simulink model "hrg_tdm_residual_observer"  (R2025a)
settings: Solver=FixedStepDiscrete  StartTime=0.0  StopTime=0  FixedStep=1  RelTol=1e-3
model workspace (MAT data in the model file):
  obs.sampleCount = 1600
  obs.jointCarrierMap = [-0.00025765079673 -0.000416664414145 -0.000202686971327 -0.000334156912121 -0.000153535532759 -0.00025977175969 -0.00010978152307 -0.000192965109295 -7.10329454025e-05 -0.000133221632945 -3.69196965297e-05 -8.00532519635e-05 ... (3200 elements, 2x1600)]
  obs.lateCarrierMap = [0 0 0 0 0 0 0 0 0 0 0 0 ... (3200 elements, 2x1600)]
  obs.holdoutErrorMap = [-0.162387616405 -0.0989965810095 -0.0526141659259 -0.0196686023406 0.00277754819147 0.0171274479295 0.0253355675884 0.0289807611935 0.0293285386507 0.027384022459 0.0239368813756 0.0195993643707 ... (640000 elements, 400x1600)]
  obs.holdoutCount = 400
  obs.holdoutMean = [0.0025 0.0025 0.0025 0.0025 0.0025 0.0025 0.0025 0.0025 0.0025 0.0025 0.0025 0.0025 ... (400 elements, 1x400)]
  obs.allMask = [1 1 1 1 1 1 1 1 1 1 1 1 ... (1600 elements, 1x1600)]
  obs.lateMask = [0 0 0 0 0 0 0 0 0 0 0 0 ... (1600 elements, 1x1600)]
  obs.jointDesignOK = 1
  obs.lateDesignOK = 1
  obs.holdoutLimit = 0.00220536539639
Description:
  | 原生分时残差观测器，1600 个样本/帧，留出 RMS 门限 0.00220537 V。
settings Model: Creator=Administrator  LastModifiedBy=Administrator
settings DataIOCC: SaveTime=off

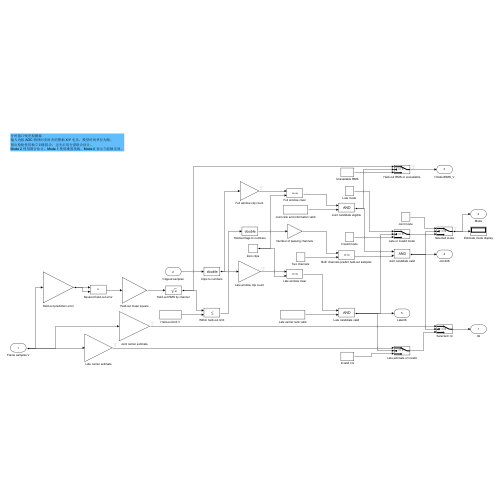
[thumbnail: Simulink's stored preview of the top-level diagram]
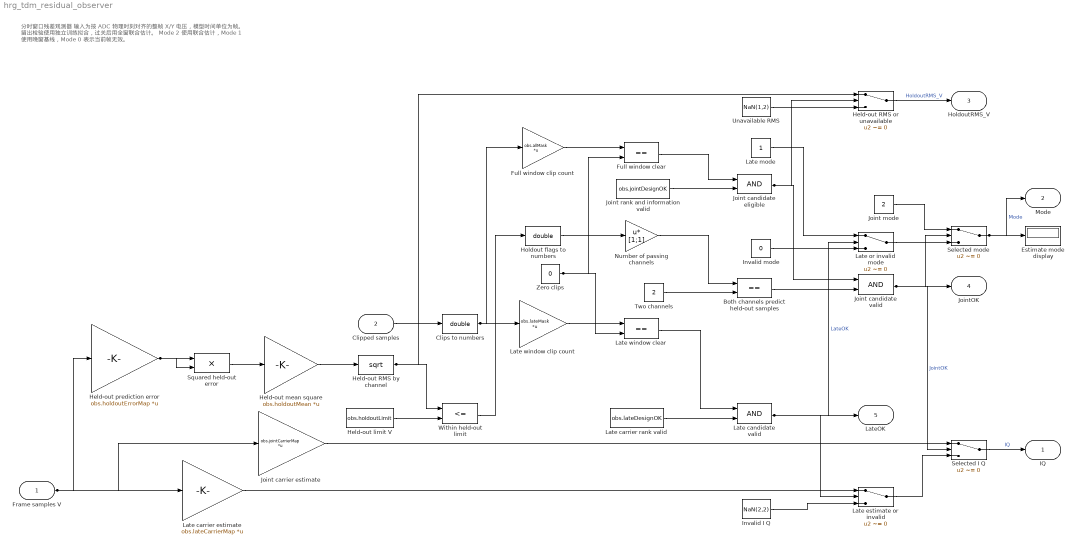
== system hrg_tdm_residual_observer ==
  note: 分时窗口残差观测器
      | 输入为按 ADC 物理时刻对齐的整帧 X/Y 电压，模型时间单位为帧。
      | 留出检验使用独立训练拟合，过关后用全窗联合估计。
      | Mode 2 使用联合估计，Mode 1 使用晚窗基线，Mode 0 表示当前帧无效。
  Frame samples V : Inport  OutDataTypeStr=double  PortDimensions=[obs.sampleCount 2]  SampleTime=1
  Clipped samples : Inport  Port=2  OutDataTypeStr=boolean  PortDimensions=obs.sampleCount  SampleTime=1
  Both channels predict held-out samples : RelationalOperator  Operator===  OutDataTypeStr=boolean  RndMeth=Simplest  InputSameDT=off
  Clips to numbers : DataTypeConversion  OutDataTypeStr=double  SaturateOnIntegerOverflow=off  RndMeth=Floor
  Estimate mode display : Display
  Full window clear : RelationalOperator  Operator===  OutDataTypeStr=boolean  RndMeth=Simplest  InputSameDT=off
  Full window clip count : Gain  Gain=obs.allMask  Multiplication=Matrix(K*u)
  Held-out RMS by channel : Math  Operator=sqrt
  Held-out RMS or unavailable : Switch  Criteria=u2 ~= 0  SaturateOnIntegerOverflow=off  InputSameDT=off
  Held-out limit V : Constant  Value=obs.holdoutLimit
  Held-out mean square : Gain  Gain=obs.holdoutMean  Multiplication=Matrix(K*u)
  Held-out prediction error : Gain  Gain=obs.holdoutErrorMap  Multiplication=Matrix(K*u)
  Holdout flags to numbers : DataTypeConversion  OutDataTypeStr=double  SaturateOnIntegerOverflow=off  RndMeth=Floor
  Invalid I Q : Constant  Value=NaN(2,2)
  Invalid mode : Constant  Value=0
  Joint candidate eligible : Logic  AllPortsSameDT=off  OutDataTypeStr=boolean
  Joint candidate valid : Logic  AllPortsSameDT=off  OutDataTypeStr=boolean
  Joint carrier estimate : Gain  Gain=obs.jointCarrierMap  Multiplication=Matrix(K*u)
  Joint mode : Constant  Value=2
  Joint rank and information valid : Constant  Value=obs.jointDesignOK
  Late candidate valid : Logic  AllPortsSameDT=off  OutDataTypeStr=boolean
  Late carrier estimate : Gain  Gain=obs.lateCarrierMap  Multiplication=Matrix(K*u)
  Late carrier rank valid : Constant  Value=obs.lateDesignOK
  Late estimate or invalid : Switch  Criteria=u2 ~= 0  SaturateOnIntegerOverflow=off  InputSameDT=off
  Late mode : Constant
  Late or invalid mode : Switch  Criteria=u2 ~= 0  SaturateOnIntegerOverflow=off  InputSameDT=off
  Late window clear : RelationalOperator  Operator===  OutDataTypeStr=boolean  RndMeth=Simplest  InputSameDT=off
  Late window clip count : Gain  Gain=obs.lateMask  Multiplication=Matrix(K*u)
  Number of passing channels : Gain  Gain=[1;1]  Multiplication=Matrix(u*K)
  Selected I Q : Switch  Criteria=u2 ~= 0  SaturateOnIntegerOverflow=off  InputSameDT=off
  Selected mode : Switch  Criteria=u2 ~= 0  SaturateOnIntegerOverflow=off  InputSameDT=off
  Squared held-out error : Product  Inputs=**
  Two channels : Constant  Value=2
  Unavailable RMS : Constant  Value=NaN(1,2)
  Within held-out limit : RelationalOperator  Operator=<=  OutDataTypeStr=boolean  RndMeth=Simplest  InputSameDT=off
  Zero clips : Constant  Value=0
  IQ : Outport
  Mode : Outport  Port=2
  HoldoutRMS_V : Outport  Port=3
  JointOK : Outport  Port=4
  LateOK : Outport  Port=5
  wires:
  Invalid I Q/1 -> Late estimate or invalid/3
  Frame samples V/1 -> Joint carrier estimate/1, Late carrier estimate/1, Held-out prediction error/1
  Late candidate valid/1 -> Late estimate or invalid/2, Late or invalid mode/2, LateOK/1  "LateOK"
  Clipped samples/1 -> Clips to numbers/1
  Held-out prediction error/1 -> Squared held-out error/2, Squared held-out error/1
  Squared held-out error/1 -> Held-out mean square/1
  Holdout flags to numbers/1 -> Number of passing channels/1
  Full window clip count/1 -> Full window clear/1
  Late carrier estimate/1 -> Late estimate or invalid/1
  Held-out mean square/1 -> Held-out RMS by channel/1
  Number of passing channels/1 -> Both channels predict held-out samples/1
  Held-out RMS by channel/1 -> Held-out RMS or unavailable/1, Within held-out limit/1
  Joint candidate eligible/1 -> Joint candidate valid/1, Held-out RMS or unavailable/2
  Full window clear/1 -> Joint candidate eligible/1
  Joint carrier estimate/1 -> Selected I Q/1
  Held-out limit V/1 -> Within held-out limit/2
  Clips to numbers/1 -> Full window clip count/1, Late window clip count/1
  Within held-out limit/1 -> Holdout flags to numbers/1
  Zero clips/1 -> Late window clear/2, Full window clear/2
  Late window clip count/1 -> Late window clear/1
  Joint rank and information valid/1 -> Joint candidate eligible/2
  Two channels/1 -> Both channels predict held-out samples/2
  Late window clear/1 -> Late candidate valid/1
  Late carrier rank valid/1 -> Late candidate valid/2
  Unavailable RMS/1 -> Held-out RMS or unavailable/3
  Late mode/1 -> Late or invalid mode/1
  Invalid mode/1 -> Late or invalid mode/3
  Both channels predict held-out samples/1 -> Joint candidate valid/2
  Held-out RMS or unavailable/1 -> HoldoutRMS_V/1  "HoldoutRMS_V"
  Joint mode/1 -> Selected mode/1
  Joint candidate valid/1 -> Selected I Q/2, Selected mode/2, JointOK/1  "JointOK"
  Late or invalid mode/1 -> Selected mode/3
  Late estimate or invalid/1 -> Selected I Q/3
  Selected mode/1 -> Mode/1, Estimate mode display/1  "Mode"
  Selected I Q/1 -> IQ/1  "IQ"
